simulink model "snap_sys_clk_feng"  (R2019a)
settings: Solver=VariableStepDiscrete  StartTime=0.0  StopTime=10.0  RelTol=1e-3
undefined symbols (not defined in the file): datetime, posixtime
libraries: xbsIndex_r4 x5252, casper_library_misc x69, xps_library x6, casper_library_delays x3
(part 12 of 45)

== system snap_sys_clk_feng/stats/calc_adc_sum_sq10 ==
  note: 127^2 == 16129
  in : Inport
  Accumulator : xbsIndex_r4/Accumulator  operation=Add  n_bits=32  overflow=Wrap  scale=1  rst=on  hasbypass=on  infoeditControl=reset for floating point data type must be asserted for a minimum of 2 cycles  en=off  latency=1  msb_inp=100  msb=100  lsb=-100  use_behavioral_HDL=on  implementation=Fabric  dbl_ovrd=off  block_type=accum
      settings: xl_area=[0, 0, 0, 0, 0, 0, 0]  block_version=10.1.3
  Accumulator1 : xbsIndex_r4/Accumulator  operation=Add  n_bits=32  overflow=Wrap  scale=1  rst=on  hasbypass=on  infoeditControl=reset for floating point data type must be asserted for a minimum of 2 cycles  en=off  latency=1  msb_inp=100  msb=100  lsb=-100  use_behavioral_HDL=on  implementation=Fabric  dbl_ovrd=off  block_type=accum
      settings: xl_area=[0, 0, 0, 0, 0, 0, 0]  block_version=10.1.3
  Accumulator2 : xbsIndex_r4/Accumulator  operation=Add  n_bits=32  overflow=Wrap  scale=1  rst=on  hasbypass=on  infoeditControl=reset for floating point data type must be asserted for a minimum of 2 cycles  en=off  latency=1  msb_inp=100  msb=100  lsb=-100  use_behavioral_HDL=on  implementation=Fabric  dbl_ovrd=off  block_type=accum
      settings: xl_area=[0, 0, 0, 0, 0, 0, 0]  block_version=10.1.3
  BitBasher : xbsIndex_r4/BitBasher  bitexpr=sss={clip, s, ss}  display_expr=off  sr_1=sss  arith_type1="Signed  (2's comp)"  bin_pt1=0  sr_2=2  arith_type2=Unsigned  bin_pt2=0  sr_3=3  arith_type3=Unsigned  bin_pt3=0  sr_4=4  arith_type4=Unsigned  bin_pt4=0  dbl_ovrd=off  block_type=bitbasher
      settings: block_version=10.1.3
  Constant : xbsIndex_r4/Constant  const=127^2  gui_display_data_type=Fixed-point  arith_type=Unsigned  n_bits=15  bin_pt=0  preci_type=Single  exp_width=8  frac_width=24  explicit_period=on  period=1  equ=P=C  opselect=C  inp2=PCIN>>17  opr=+  inp1=P  carry=CIN  dbl_ovrd=off  block_type=constant
  Delay : xbsIndex_r4/Delay  rst=off  infoeditControl=Selection of Reset will increase slice count due to use of real FFs and instead of SRLs  en=off  latency=2  reg_retiming=off  dbl_ovrd=off  block_type=delay
  Delay1 : xbsIndex_r4/Delay  rst=off  infoeditControl=Selection of Reset will increase slice count due to use of real FFs and instead of SRLs  en=off  latency=1  reg_retiming=off  dbl_ovrd=off  block_type=delay
  Delay2 : xbsIndex_r4/Delay  rst=off  infoeditControl=Selection of Reset will increase slice count due to use of real FFs and instead of SRLs  en=off  latency=1  reg_retiming=off  dbl_ovrd=off  block_type=delay
      settings: infoedit=Hardware notes: A delay line is a chain, each link of which is an SRL16 or SRL32 followed by a flip-flop.
  Mult : xbsIndex_r4/Mult  precision=User Defined  arith_type=Unsigned  n_bits=15  bin_pt=0  quantization=Truncate  overflow=Wrap  en=off  latency=2  use_behavioral_HDL=on  opt=Speed  use_embedded=on  optimum_pipeline=on  pipeline=on  dbl_ovrd=off  use_rpm=on  placement_style=Rectangular shape  block_type=mult
      settings: xl_area=[0, 0, 0, 0, 0, 0, 0]  block_version=10.1.3
  Register : xbsIndex_r4/Register  init=0  rst=off  en=on  dbl_ovrd=off  block_type=register
      settings: xl_area=[0, 0, 0, 0, 0, 0, 0]
  Register1 : xbsIndex_r4/Register  init=0  rst=off  en=on  dbl_ovrd=off  block_type=register
      settings: xl_area=[0, 0, 0, 0, 0, 0, 0]
  Register2 : xbsIndex_r4/Register  init=0  rst=off  en=on  dbl_ovrd=off  block_type=register
      settings: xl_area=[0, 0, 0, 0, 0, 0, 0]
  Reinterpret : xbsIndex_r4/Reinterpret  force_arith_type=off  arith_type=Unsigned  force_bin_pt=on  bin_pt=0  block_type=reinterpret
  Relational : xbsIndex_r4/Relational  mode=a>=b  op_type=Ufix  en=off  latency=0  dbl_ovrd=off  block_type=relational
  sum_sumsq : Outport
  wires:
  in/1 -> Reinterpret/1
  [adc_rms_rst] -> Delay2/1
  Accumulator/1 -> Register/1
  Mult/1 -> Accumulator/1, Relational/1
  Accumulator1/1 -> Register1/1
  Delay/1 -> Accumulator1/1
  BitBasher/1 -> sum_sumsq/1
  Delay1/1 -> Mult/2, Mult/1, Delay/1
  Reinterpret/1 -> Delay1/1
  Constant/1 -> Relational/2
  Relational/1 -> Accumulator2/1
  Delay2/1 -> Accumulator2/2, Accumulator1/2, Accumulator/2, Register2/2, Register1/2, Register/2
  Accumulator2/1 -> Register2/1
  Register1/1 -> BitBasher/2
  Register/1 -> BitBasher/3
  Register2/1 -> BitBasher/1

== system snap_sys_clk_feng/stats/calc_adc_sum_sq11 ==
  note: 127^2 == 16129
  in : Inport
  Accumulator : xbsIndex_r4/Accumulator  operation=Add  n_bits=32  overflow=Wrap  scale=1  rst=on  hasbypass=on  infoeditControl=reset for floating point data type must be asserted for a minimum of 2 cycles  en=off  latency=1  msb_inp=100  msb=100  lsb=-100  use_behavioral_HDL=on  implementation=Fabric  dbl_ovrd=off  block_type=accum
      settings: xl_area=[0, 0, 0, 0, 0, 0, 0]  block_version=10.1.3
  Accumulator1 : xbsIndex_r4/Accumulator  operation=Add  n_bits=32  overflow=Wrap  scale=1  rst=on  hasbypass=on  infoeditControl=reset for floating point data type must be asserted for a minimum of 2 cycles  en=off  latency=1  msb_inp=100  msb=100  lsb=-100  use_behavioral_HDL=on  implementation=Fabric  dbl_ovrd=off  block_type=accum
      settings: xl_area=[0, 0, 0, 0, 0, 0, 0]  block_version=10.1.3
  Accumulator2 : xbsIndex_r4/Accumulator  operation=Add  n_bits=32  overflow=Wrap  scale=1  rst=on  hasbypass=on  infoeditControl=reset for floating point data type must be asserted for a minimum of 2 cycles  en=off  latency=1  msb_inp=100  msb=100  lsb=-100  use_behavioral_HDL=on  implementation=Fabric  dbl_ovrd=off  block_type=accum
      settings: xl_area=[0, 0, 0, 0, 0, 0, 0]  block_version=10.1.3
  BitBasher : xbsIndex_r4/BitBasher  bitexpr=sss={clip, s, ss}  display_expr=off  sr_1=sss  arith_type1="Signed  (2's comp)"  bin_pt1=0  sr_2=2  arith_type2=Unsigned  bin_pt2=0  sr_3=3  arith_type3=Unsigned  bin_pt3=0  sr_4=4  arith_type4=Unsigned  bin_pt4=0  dbl_ovrd=off  block_type=bitbasher
      settings: block_version=10.1.3
  Constant : xbsIndex_r4/Constant  const=127^2  gui_display_data_type=Fixed-point  arith_type=Unsigned  n_bits=15  bin_pt=0  preci_type=Single  exp_width=8  frac_width=24  explicit_period=on  period=1  equ=P=C  opselect=C  inp2=PCIN>>17  opr=+  inp1=P  carry=CIN  dbl_ovrd=off  block_type=constant
  Delay : xbsIndex_r4/Delay  rst=off  infoeditControl=Selection of Reset will increase slice count due to use of real FFs and instead of SRLs  en=off  latency=2  reg_retiming=off  dbl_ovrd=off  block_type=delay
  Delay1 : xbsIndex_r4/Delay  rst=off  infoeditControl=Selection of Reset will increase slice count due to use of real FFs and instead of SRLs  en=off  latency=1  reg_retiming=off  dbl_ovrd=off  block_type=delay
  Delay2 : xbsIndex_r4/Delay  rst=off  infoeditControl=Selection of Reset will increase slice count due to use of real FFs and instead of SRLs  en=off  latency=1  reg_retiming=off  dbl_ovrd=off  block_type=delay
      settings: infoedit=Hardware notes: A delay line is a chain, each link of which is an SRL16 or SRL32 followed by a flip-flop.
  Mult : xbsIndex_r4/Mult  precision=User Defined  arith_type=Unsigned  n_bits=15  bin_pt=0  quantization=Truncate  overflow=Wrap  en=off  latency=2  use_behavioral_HDL=on  opt=Speed  use_embedded=on  optimum_pipeline=on  pipeline=on  dbl_ovrd=off  use_rpm=on  placement_style=Rectangular shape  block_type=mult
      settings: xl_area=[0, 0, 0, 0, 0, 0, 0]  block_version=10.1.3
  Register : xbsIndex_r4/Register  init=0  rst=off  en=on  dbl_ovrd=off  block_type=register
      settings: xl_area=[0, 0, 0, 0, 0, 0, 0]
  Register1 : xbsIndex_r4/Register  init=0  rst=off  en=on  dbl_ovrd=off  block_type=register
      settings: xl_area=[0, 0, 0, 0, 0, 0, 0]
  Register2 : xbsIndex_r4/Register  init=0  rst=off  en=on  dbl_ovrd=off  block_type=register
      settings: xl_area=[0, 0, 0, 0, 0, 0, 0]
  Reinterpret : xbsIndex_r4/Reinterpret  force_arith_type=off  arith_type=Unsigned  force_bin_pt=on  bin_pt=0  block_type=reinterpret
  Relational : xbsIndex_r4/Relational  mode=a>=b  op_type=Ufix  en=off  latency=0  dbl_ovrd=off  block_type=relational
  sum_sumsq : Outport
  wires:
  Register2/1 -> BitBasher/1
  Register/1 -> BitBasher/3
  Register1/1 -> BitBasher/2
  Accumulator2/1 -> Register2/1
  Delay2/1 -> Register/2, Register1/2, Register2/2, Accumulator/2, Accumulator1/2, Accumulator2/2
  Relational/1 -> Accumulator2/1
  Constant/1 -> Relational/2
  Reinterpret/1 -> Delay1/1
  Delay1/1 -> Delay/1, Mult/1, Mult/2
  BitBasher/1 -> sum_sumsq/1
  Delay/1 -> Accumulator1/1
  Accumulator1/1 -> Register1/1
  Mult/1 -> Relational/1, Accumulator/1
  Accumulator/1 -> Register/1
  [adc_rms_rst] -> Delay2/1
  in/1 -> Reinterpret/1

== system snap_sys_clk_feng/stats/calc_adc_sum_sq12 ==
  note: 127^2 == 16129
  in : Inport
  Accumulator : xbsIndex_r4/Accumulator  operation=Add  n_bits=32  overflow=Wrap  scale=1  rst=on  hasbypass=on  infoeditControl=reset for floating point data type must be asserted for a minimum of 2 cycles  en=off  latency=1  msb_inp=100  msb=100  lsb=-100  use_behavioral_HDL=on  implementation=Fabric  dbl_ovrd=off  block_type=accum
      settings: xl_area=[0, 0, 0, 0, 0, 0, 0]  block_version=10.1.3
  Accumulator1 : xbsIndex_r4/Accumulator  operation=Add  n_bits=32  overflow=Wrap  scale=1  rst=on  hasbypass=on  infoeditControl=reset for floating point data type must be asserted for a minimum of 2 cycles  en=off  latency=1  msb_inp=100  msb=100  lsb=-100  use_behavioral_HDL=on  implementation=Fabric  dbl_ovrd=off  block_type=accum
      settings: xl_area=[0, 0, 0, 0, 0, 0, 0]  block_version=10.1.3
  Accumulator2 : xbsIndex_r4/Accumulator  operation=Add  n_bits=32  overflow=Wrap  scale=1  rst=on  hasbypass=on  infoeditControl=reset for floating point data type must be asserted for a minimum of 2 cycles  en=off  latency=1  msb_inp=100  msb=100  lsb=-100  use_behavioral_HDL=on  implementation=Fabric  dbl_ovrd=off  block_type=accum
      settings: xl_area=[0, 0, 0, 0, 0, 0, 0]  block_version=10.1.3
  BitBasher : xbsIndex_r4/BitBasher  bitexpr=sss={clip, s, ss}  display_expr=off  sr_1=sss  arith_type1="Signed  (2's comp)"  bin_pt1=0  sr_2=2  arith_type2=Unsigned  bin_pt2=0  sr_3=3  arith_type3=Unsigned  bin_pt3=0  sr_4=4  arith_type4=Unsigned  bin_pt4=0  dbl_ovrd=off  block_type=bitbasher
      settings: block_version=10.1.3
  Constant : xbsIndex_r4/Constant  const=127^2  gui_display_data_type=Fixed-point  arith_type=Unsigned  n_bits=15  bin_pt=0  preci_type=Single  exp_width=8  frac_width=24  explicit_period=on  period=1  equ=P=C  opselect=C  inp2=PCIN>>17  opr=+  inp1=P  carry=CIN  dbl_ovrd=off  block_type=constant
  Delay : xbsIndex_r4/Delay  rst=off  infoeditControl=Selection of Reset will increase slice count due to use of real FFs and instead of SRLs  en=off  latency=2  reg_retiming=off  dbl_ovrd=off  block_type=delay
  Delay1 : xbsIndex_r4/Delay  rst=off  infoeditControl=Selection of Reset will increase slice count due to use of real FFs and instead of SRLs  en=off  latency=1  reg_retiming=off  dbl_ovrd=off  block_type=delay
  Delay2 : xbsIndex_r4/Delay  rst=off  infoeditControl=Selection of Reset will increase slice count due to use of real FFs and instead of SRLs  en=off  latency=1  reg_retiming=off  dbl_ovrd=off  block_type=delay
      settings: infoedit=Hardware notes: A delay line is a chain, each link of which is an SRL16 or SRL32 followed by a flip-flop.
  Mult : xbsIndex_r4/Mult  precision=User Defined  arith_type=Unsigned  n_bits=15  bin_pt=0  quantization=Truncate  overflow=Wrap  en=off  latency=2  use_behavioral_HDL=on  opt=Speed  use_embedded=on  optimum_pipeline=on  pipeline=on  dbl_ovrd=off  use_rpm=on  placement_style=Rectangular shape  block_type=mult
      settings: xl_area=[0, 0, 0, 0, 0, 0, 0]  block_version=10.1.3
  Register : xbsIndex_r4/Register  init=0  rst=off  en=on  dbl_ovrd=off  block_type=register
      settings: xl_area=[0, 0, 0, 0, 0, 0, 0]
  Register1 : xbsIndex_r4/Register  init=0  rst=off  en=on  dbl_ovrd=off  block_type=register
      settings: xl_area=[0, 0, 0, 0, 0, 0, 0]
  Register2 : xbsIndex_r4/Register  init=0  rst=off  en=on  dbl_ovrd=off  block_type=register
      settings: xl_area=[0, 0, 0, 0, 0, 0, 0]
  Reinterpret : xbsIndex_r4/Reinterpret  force_arith_type=off  arith_type=Unsigned  force_bin_pt=on  bin_pt=0  block_type=reinterpret
  Relational : xbsIndex_r4/Relational  mode=a>=b  op_type=Ufix  en=off  latency=0  dbl_ovrd=off  block_type=relational
  sum_sumsq : Outport
  wires:
  in/1 -> Reinterpret/1
  [adc_rms_rst] -> Delay2/1
  Accumulator/1 -> Register/1
  Mult/1 -> Accumulator/1, Relational/1
  Accumulator1/1 -> Register1/1
  Delay/1 -> Accumulator1/1
  BitBasher/1 -> sum_sumsq/1
  Delay1/1 -> Mult/2, Mult/1, Delay/1
  Reinterpret/1 -> Delay1/1
  Constant/1 -> Relational/2
  Relational/1 -> Accumulator2/1
  Delay2/1 -> Accumulator2/2, Accumulator1/2, Accumulator/2, Register2/2, Register1/2, Register/2
  Accumulator2/1 -> Register2/1
  Register1/1 -> BitBasher/2
  Register/1 -> BitBasher/3
  Register2/1 -> BitBasher/1

== system snap_sys_clk_feng/stats/calc_adc_sum_sq13 ==
  note: 127^2 == 16129
  in : Inport
  Accumulator : xbsIndex_r4/Accumulator  operation=Add  n_bits=32  overflow=Wrap  scale=1  rst=on  hasbypass=on  infoeditControl=reset for floating point data type must be asserted for a minimum of 2 cycles  en=off  latency=1  msb_inp=100  msb=100  lsb=-100  use_behavioral_HDL=on  implementation=Fabric  dbl_ovrd=off  block_type=accum
      settings: xl_area=[0, 0, 0, 0, 0, 0, 0]  block_version=10.1.3
  Accumulator1 : xbsIndex_r4/Accumulator  operation=Add  n_bits=32  overflow=Wrap  scale=1  rst=on  hasbypass=on  infoeditControl=reset for floating point data type must be asserted for a minimum of 2 cycles  en=off  latency=1  msb_inp=100  msb=100  lsb=-100  use_behavioral_HDL=on  implementation=Fabric  dbl_ovrd=off  block_type=accum
      settings: xl_area=[0, 0, 0, 0, 0, 0, 0]  block_version=10.1.3
  Accumulator2 : xbsIndex_r4/Accumulator  operation=Add  n_bits=32  overflow=Wrap  scale=1  rst=on  hasbypass=on  infoeditControl=reset for floating point data type must be asserted for a minimum of 2 cycles  en=off  latency=1  msb_inp=100  msb=100  lsb=-100  use_behavioral_HDL=on  implementation=Fabric  dbl_ovrd=off  block_type=accum
      settings: xl_area=[0, 0, 0, 0, 0, 0, 0]  block_version=10.1.3
  BitBasher : xbsIndex_r4/BitBasher  bitexpr=sss={clip, s, ss}  display_expr=off  sr_1=sss  arith_type1="Signed  (2's comp)"  bin_pt1=0  sr_2=2  arith_type2=Unsigned  bin_pt2=0  sr_3=3  arith_type3=Unsigned  bin_pt3=0  sr_4=4  arith_type4=Unsigned  bin_pt4=0  dbl_ovrd=off  block_type=bitbasher
      settings: block_version=10.1.3
  Constant : xbsIndex_r4/Constant  const=127^2  gui_display_data_type=Fixed-point  arith_type=Unsigned  n_bits=15  bin_pt=0  preci_type=Single  exp_width=8  frac_width=24  explicit_period=on  period=1  equ=P=C  opselect=C  inp2=PCIN>>17  opr=+  inp1=P  carry=CIN  dbl_ovrd=off  block_type=constant
  Delay : xbsIndex_r4/Delay  rst=off  infoeditControl=Selection of Reset will increase slice count due to use of real FFs and instead of SRLs  en=off  latency=2  reg_retiming=off  dbl_ovrd=off  block_type=delay
  Delay1 : xbsIndex_r4/Delay  rst=off  infoeditControl=Selection of Reset will increase slice count due to use of real FFs and instead of SRLs  en=off  latency=1  reg_retiming=off  dbl_ovrd=off  block_type=delay
  Delay2 : xbsIndex_r4/Delay  rst=off  infoeditControl=Selection of Reset will increase slice count due to use of real FFs and instead of SRLs  en=off  latency=1  reg_retiming=off  dbl_ovrd=off  block_type=delay
      settings: infoedit=Hardware notes: A delay line is a chain, each link of which is an SRL16 or SRL32 followed by a flip-flop.
  Mult : xbsIndex_r4/Mult  precision=User Defined  arith_type=Unsigned  n_bits=15  bin_pt=0  quantization=Truncate  overflow=Wrap  en=off  latency=2  use_behavioral_HDL=on  opt=Speed  use_embedded=on  optimum_pipeline=on  pipeline=on  dbl_ovrd=off  use_rpm=on  placement_style=Rectangular shape  block_type=mult
      settings: xl_area=[0, 0, 0, 0, 0, 0, 0]  block_version=10.1.3
  Register : xbsIndex_r4/Register  init=0  rst=off  en=on  dbl_ovrd=off  block_type=register
      settings: xl_area=[0, 0, 0, 0, 0, 0, 0]
  Register1 : xbsIndex_r4/Register  init=0  rst=off  en=on  dbl_ovrd=off  block_type=register
      settings: xl_area=[0, 0, 0, 0, 0, 0, 0]
  Register2 : xbsIndex_r4/Register  init=0  rst=off  en=on  dbl_ovrd=off  block_type=register
      settings: xl_area=[0, 0, 0, 0, 0, 0, 0]
  Reinterpret : xbsIndex_r4/Reinterpret  force_arith_type=off  arith_type=Unsigned  force_bin_pt=on  bin_pt=0  block_type=reinterpret
  Relational : xbsIndex_r4/Relational  mode=a>=b  op_type=Ufix  en=off  latency=0  dbl_ovrd=off  block_type=relational
  sum_sumsq : Outport
  wires:
  Register2/1 -> BitBasher/1
  Register/1 -> BitBasher/3
  Register1/1 -> BitBasher/2
  Accumulator2/1 -> Register2/1
  Delay2/1 -> Register/2, Register1/2, Register2/2, Accumulator/2, Accumulator1/2, Accumulator2/2
  Relational/1 -> Accumulator2/1
  Constant/1 -> Relational/2
  Reinterpret/1 -> Delay1/1
  Delay1/1 -> Delay/1, Mult/1, Mult/2
  BitBasher/1 -> sum_sumsq/1
  Delay/1 -> Accumulator1/1
  Accumulator1/1 -> Register1/1
  Mult/1 -> Relational/1, Accumulator/1
  Accumulator/1 -> Register/1
  [adc_rms_rst] -> Delay2/1
  in/1 -> Reinterpret/1

== system snap_sys_clk_feng/stats/calc_adc_sum_sq14 ==
  note: 127^2 == 16129
  in : Inport
  Accumulator : xbsIndex_r4/Accumulator  operation=Add  n_bits=32  overflow=Wrap  scale=1  rst=on  hasbypass=on  infoeditControl=reset for floating point data type must be asserted for a minimum of 2 cycles  en=off  latency=1  msb_inp=100  msb=100  lsb=-100  use_behavioral_HDL=on  implementation=Fabric  dbl_ovrd=off  block_type=accum
      settings: xl_area=[0, 0, 0, 0, 0, 0, 0]  block_version=10.1.3
  Accumulator1 : xbsIndex_r4/Accumulator  operation=Add  n_bits=32  overflow=Wrap  scale=1  rst=on  hasbypass=on  infoeditControl=reset for floating point data type must be asserted for a minimum of 2 cycles  en=off  latency=1  msb_inp=100  msb=100  lsb=-100  use_behavioral_HDL=on  implementation=Fabric  dbl_ovrd=off  block_type=accum
      settings: xl_area=[0, 0, 0, 0, 0, 0, 0]  block_version=10.1.3
  Accumulator2 : xbsIndex_r4/Accumulator  operation=Add  n_bits=32  overflow=Wrap  scale=1  rst=on  hasbypass=on  infoeditControl=reset for floating point data type must be asserted for a minimum of 2 cycles  en=off  latency=1  msb_inp=100  msb=100  lsb=-100  use_behavioral_HDL=on  implementation=Fabric  dbl_ovrd=off  block_type=accum
      settings: xl_area=[0, 0, 0, 0, 0, 0, 0]  block_version=10.1.3
  BitBasher : xbsIndex_r4/BitBasher  bitexpr=sss={clip, s, ss}  display_expr=off  sr_1=sss  arith_type1="Signed  (2's comp)"  bin_pt1=0  sr_2=2  arith_type2=Unsigned  bin_pt2=0  sr_3=3  arith_type3=Unsigned  bin_pt3=0  sr_4=4  arith_type4=Unsigned  bin_pt4=0  dbl_ovrd=off  block_type=bitbasher
      settings: block_version=10.1.3
  Constant : xbsIndex_r4/Constant  const=127^2  gui_display_data_type=Fixed-point  arith_type=Unsigned  n_bits=15  bin_pt=0  preci_type=Single  exp_width=8  frac_width=24  explicit_period=on  period=1  equ=P=C  opselect=C  inp2=PCIN>>17  opr=+  inp1=P  carry=CIN  dbl_ovrd=off  block_type=constant
  Delay : xbsIndex_r4/Delay  rst=off  infoeditControl=Selection of Reset will increase slice count due to use of real FFs and instead of SRLs  en=off  latency=2  reg_retiming=off  dbl_ovrd=off  block_type=delay
  Delay1 : xbsIndex_r4/Delay  rst=off  infoeditControl=Selection of Reset will increase slice count due to use of real FFs and instead of SRLs  en=off  latency=1  reg_retiming=off  dbl_ovrd=off  block_type=delay
  Delay2 : xbsIndex_r4/Delay  rst=off  infoeditControl=Selection of Reset will increase slice count due to use of real FFs and instead of SRLs  en=off  latency=1  reg_retiming=off  dbl_ovrd=off  block_type=delay
      settings: infoedit=Hardware notes: A delay line is a chain, each link of which is an SRL16 or SRL32 followed by a flip-flop.
  Mult : xbsIndex_r4/Mult  precision=User Defined  arith_type=Unsigned  n_bits=15  bin_pt=0  quantization=Truncate  overflow=Wrap  en=off  latency=2  use_behavioral_HDL=on  opt=Speed  use_embedded=on  optimum_pipeline=on  pipeline=on  dbl_ovrd=off  use_rpm=on  placement_style=Rectangular shape  block_type=mult
      settings: xl_area=[0, 0, 0, 0, 0, 0, 0]  block_version=10.1.3
  Register : xbsIndex_r4/Register  init=0  rst=off  en=on  dbl_ovrd=off  block_type=register
      settings: xl_area=[0, 0, 0, 0, 0, 0, 0]
  Register1 : xbsIndex_r4/Register  init=0  rst=off  en=on  dbl_ovrd=off  block_type=register
      settings: xl_area=[0, 0, 0, 0, 0, 0, 0]
  Register2 : xbsIndex_r4/Register  init=0  rst=off  en=on  dbl_ovrd=off  block_type=register
      settings: xl_area=[0, 0, 0, 0, 0, 0, 0]
  Reinterpret : xbsIndex_r4/Reinterpret  force_arith_type=off  arith_type=Unsigned  force_bin_pt=on  bin_pt=0  block_type=reinterpret
  Relational : xbsIndex_r4/Relational  mode=a>=b  op_type=Ufix  en=off  latency=0  dbl_ovrd=off  block_type=relational
  sum_sumsq : Outport
  wires:
  Register2/1 -> BitBasher/1
  Register/1 -> BitBasher/3
  Register1/1 -> BitBasher/2
  Accumulator2/1 -> Register2/1
  Delay2/1 -> Register/2, Register1/2, Register2/2, Accumulator/2, Accumulator1/2, Accumulator2/2
  Relational/1 -> Accumulator2/1
  Constant/1 -> Relational/2
  Reinterpret/1 -> Delay1/1
  Delay1/1 -> Delay/1, Mult/1, Mult/2
  BitBasher/1 -> sum_sumsq/1
  Delay/1 -> Accumulator1/1
  Accumulator1/1 -> Register1/1
  Mult/1 -> Relational/1, Accumulator/1
  Accumulator/1 -> Register/1
  [adc_rms_rst] -> Delay2/1
  in/1 -> Reinterpret/1

== system snap_sys_clk_feng/stats/calc_adc_sum_sq15 ==
  note: 127^2 == 16129
  in : Inport
  Accumulator : xbsIndex_r4/Accumulator  operation=Add  n_bits=32  overflow=Wrap  scale=1  rst=on  hasbypass=on  infoeditControl=reset for floating point data type must be asserted for a minimum of 2 cycles  en=off  latency=1  msb_inp=100  msb=100  lsb=-100  use_behavioral_HDL=on  implementation=Fabric  dbl_ovrd=off  block_type=accum
      settings: xl_area=[0, 0, 0, 0, 0, 0, 0]  block_version=10.1.3
  Accumulator1 : xbsIndex_r4/Accumulator  operation=Add  n_bits=32  overflow=Wrap  scale=1  rst=on  hasbypass=on  infoeditControl=reset for floating point data type must be asserted for a minimum of 2 cycles  en=off  latency=1  msb_inp=100  msb=100  lsb=-100  use_behavioral_HDL=on  implementation=Fabric  dbl_ovrd=off  block_type=accum
      settings: xl_area=[0, 0, 0, 0, 0, 0, 0]  block_version=10.1.3
  Accumulator2 : xbsIndex_r4/Accumulator  operation=Add  n_bits=32  overflow=Wrap  scale=1  rst=on  hasbypass=on  infoeditControl=reset for floating point data type must be asserted for a minimum of 2 cycles  en=off  latency=1  msb_inp=100  msb=100  lsb=-100  use_behavioral_HDL=on  implementation=Fabric  dbl_ovrd=off  block_type=accum
      settings: xl_area=[0, 0, 0, 0, 0, 0, 0]  block_version=10.1.3
  BitBasher : xbsIndex_r4/BitBasher  bitexpr=sss={clip, s, ss}  display_expr=off  sr_1=sss  arith_type1="Signed  (2's comp)"  bin_pt1=0  sr_2=2  arith_type2=Unsigned  bin_pt2=0  sr_3=3  arith_type3=Unsigned  bin_pt3=0  sr_4=4  arith_type4=Unsigned  bin_pt4=0  dbl_ovrd=off  block_type=bitbasher
      settings: block_version=10.1.3
  Constant : xbsIndex_r4/Constant  const=127^2  gui_display_data_type=Fixed-point  arith_type=Unsigned  n_bits=15  bin_pt=0  preci_type=Single  exp_width=8  frac_width=24  explicit_period=on  period=1  equ=P=C  opselect=C  inp2=PCIN>>17  opr=+  inp1=P  carry=CIN  dbl_ovrd=off  block_type=constant
  Delay : xbsIndex_r4/Delay  rst=off  infoeditControl=Selection of Reset will increase slice count due to use of real FFs and instead of SRLs  en=off  latency=2  reg_retiming=off  dbl_ovrd=off  block_type=delay
  Delay1 : xbsIndex_r4/Delay  rst=off  infoeditControl=Selection of Reset will increase slice count due to use of real FFs and instead of SRLs  en=off  latency=1  reg_retiming=off  dbl_ovrd=off  block_type=delay
  Delay2 : xbsIndex_r4/Delay  rst=off  infoeditControl=Selection of Reset will increase slice count due to use of real FFs and instead of SRLs  en=off  latency=1  reg_retiming=off  dbl_ovrd=off  block_type=delay
      settings: infoedit=Hardware notes: A delay line is a chain, each link of which is an SRL16 or SRL32 followed by a flip-flop.
  Mult : xbsIndex_r4/Mult  precision=User Defined  arith_type=Unsigned  n_bits=15  bin_pt=0  quantization=Truncate  overflow=Wrap  en=off  latency=2  use_behavioral_HDL=on  opt=Speed  use_embedded=on  optimum_pipeline=on  pipeline=on  dbl_ovrd=off  use_rpm=on  placement_style=Rectangular shape  block_type=mult
      settings: xl_area=[0, 0, 0, 0, 0, 0, 0]  block_version=10.1.3
  Register : xbsIndex_r4/Register  init=0  rst=off  en=on  dbl_ovrd=off  block_type=register
      settings: xl_area=[0, 0, 0, 0, 0, 0, 0]
  Register1 : xbsIndex_r4/Register  init=0  rst=off  en=on  dbl_ovrd=off  block_type=register
      settings: xl_area=[0, 0, 0, 0, 0, 0, 0]
  Register2 : xbsIndex_r4/Register  init=0  rst=off  en=on  dbl_ovrd=off  block_type=register
      settings: xl_area=[0, 0, 0, 0, 0, 0, 0]
  Reinterpret : xbsIndex_r4/Reinterpret  force_arith_type=off  arith_type=Unsigned  force_bin_pt=on  bin_pt=0  block_type=reinterpret
  Relational : xbsIndex_r4/Relational  mode=a>=b  op_type=Ufix  en=off  latency=0  dbl_ovrd=off  block_type=relational
  sum_sumsq : Outport
  wires:
  in/1 -> Reinterpret/1
  [adc_rms_rst] -> Delay2/1
  Accumulator/1 -> Register/1
  Mult/1 -> Accumulator/1, Relational/1
  Accumulator1/1 -> Register1/1
  Delay/1 -> Accumulator1/1
  BitBasher/1 -> sum_sumsq/1
  Delay1/1 -> Mult/2, Mult/1, Delay/1
  Reinterpret/1 -> Delay1/1
  Constant/1 -> Relational/2
  Relational/1 -> Accumulator2/1
  Delay2/1 -> Accumulator2/2, Accumulator1/2, Accumulator/2, Register2/2, Register1/2, Register/2
  Accumulator2/1 -> Register2/1
  Register1/1 -> BitBasher/2
  Register/1 -> BitBasher/3
  Register2/1 -> BitBasher/1

== system snap_sys_clk_feng/stats/calc_adc_sum_sq2 ==
  note: 127^2 == 16129
  in : Inport
  Accumulator : xbsIndex_r4/Accumulator  operation=Add  n_bits=32  overflow=Wrap  scale=1  rst=on  hasbypass=on  infoeditControl=reset for floating point data type must be asserted for a minimum of 2 cycles  en=off  latency=1  msb_inp=100  msb=100  lsb=-100  use_behavioral_HDL=on  implementation=Fabric  dbl_ovrd=off  block_type=accum
      settings: xl_area=[0, 0, 0, 0, 0, 0, 0]  block_version=10.1.3
  Accumulator1 : xbsIndex_r4/Accumulator  operation=Add  n_bits=32  overflow=Wrap  scale=1  rst=on  hasbypass=on  infoeditControl=reset for floating point data type must be asserted for a minimum of 2 cycles  en=off  latency=1  msb_inp=100  msb=100  lsb=-100  use_behavioral_HDL=on  implementation=Fabric  dbl_ovrd=off  block_type=accum
      settings: xl_area=[0, 0, 0, 0, 0, 0, 0]  block_version=10.1.3
  Accumulator2 : xbsIndex_r4/Accumulator  operation=Add  n_bits=32  overflow=Wrap  scale=1  rst=on  hasbypass=on  infoeditControl=reset for floating point data type must be asserted for a minimum of 2 cycles  en=off  latency=1  msb_inp=100  msb=100  lsb=-100  use_behavioral_HDL=on  implementation=Fabric  dbl_ovrd=off  block_type=accum
      settings: xl_area=[0, 0, 0, 0, 0, 0, 0]  block_version=10.1.3
  BitBasher : xbsIndex_r4/BitBasher  bitexpr=sss={clip, s, ss}  display_expr=off  sr_1=sss  arith_type1="Signed  (2's comp)"  bin_pt1=0  sr_2=2  arith_type2=Unsigned  bin_pt2=0  sr_3=3  arith_type3=Unsigned  bin_pt3=0  sr_4=4  arith_type4=Unsigned  bin_pt4=0  dbl_ovrd=off  block_type=bitbasher
      settings: block_version=10.1.3
  Constant : xbsIndex_r4/Constant  const=127^2  gui_display_data_type=Fixed-point  arith_type=Unsigned  n_bits=15  bin_pt=0  preci_type=Single  exp_width=8  frac_width=24  explicit_period=on  period=1  equ=P=C  opselect=C  inp2=PCIN>>17  opr=+  inp1=P  carry=CIN  dbl_ovrd=off  block_type=constant
  Delay : xbsIndex_r4/Delay  rst=off  infoeditControl=Selection of Reset will increase slice count due to use of real FFs and instead of SRLs  en=off  latency=2  reg_retiming=off  dbl_ovrd=off  block_type=delay
  Delay1 : xbsIndex_r4/Delay  rst=off  infoeditControl=Selection of Reset will increase slice count due to use of real FFs and instead of SRLs  en=off  latency=1  reg_retiming=off  dbl_ovrd=off  block_type=delay
  Delay2 : xbsIndex_r4/Delay  rst=off  infoeditControl=Selection of Reset will increase slice count due to use of real FFs and instead of SRLs  en=off  latency=1  reg_retiming=off  dbl_ovrd=off  block_type=delay
      settings: infoedit=Hardware notes: A delay line is a chain, each link of which is an SRL16 or SRL32 followed by a flip-flop.
  Mult : xbsIndex_r4/Mult  precision=User Defined  arith_type=Unsigned  n_bits=15  bin_pt=0  quantization=Truncate  overflow=Wrap  en=off  latency=2  use_behavioral_HDL=on  opt=Speed  use_embedded=on  optimum_pipeline=on  pipeline=on  dbl_ovrd=off  use_rpm=on  placement_style=Rectangular shape  block_type=mult
      settings: xl_area=[0, 0, 0, 0, 0, 0, 0]  block_version=10.1.3
  Register : xbsIndex_r4/Register  init=0  rst=off  en=on  dbl_ovrd=off  block_type=register
      settings: xl_area=[0, 0, 0, 0, 0, 0, 0]
  Register1 : xbsIndex_r4/Register  init=0  rst=off  en=on  dbl_ovrd=off  block_type=register
      settings: xl_area=[0, 0, 0, 0, 0, 0, 0]
  Register2 : xbsIndex_r4/Register  init=0  rst=off  en=on  dbl_ovrd=off  block_type=register
      settings: xl_area=[0, 0, 0, 0, 0, 0, 0]
  Reinterpret : xbsIndex_r4/Reinterpret  force_arith_type=off  arith_type=Unsigned  force_bin_pt=on  bin_pt=0  block_type=reinterpret
  Relational : xbsIndex_r4/Relational  mode=a>=b  op_type=Ufix  en=off  latency=0  dbl_ovrd=off  block_type=relational
  sum_sumsq : Outport
  wires:
  Register2/1 -> BitBasher/1
  Register/1 -> BitBasher/3
  Register1/1 -> BitBasher/2
  Accumulator2/1 -> Register2/1
  Delay2/1 -> Register/2, Register1/2, Register2/2, Accumulator/2, Accumulator1/2, Accumulator2/2
  Relational/1 -> Accumulator2/1
  Constant/1 -> Relational/2
  Reinterpret/1 -> Delay1/1
  Delay1/1 -> Delay/1, Mult/1, Mult/2
  BitBasher/1 -> sum_sumsq/1
  Delay/1 -> Accumulator1/1
  Accumulator1/1 -> Register1/1
  Mult/1 -> Relational/1, Accumulator/1
  Accumulator/1 -> Register/1
  [adc_rms_rst] -> Delay2/1
  in/1 -> Reinterpret/1

== system snap_sys_clk_feng/stats/calc_adc_sum_sq3 ==
  note: 127^2 == 16129
  in : Inport
  Accumulator : xbsIndex_r4/Accumulator  operation=Add  n_bits=32  overflow=Wrap  scale=1  rst=on  hasbypass=on  infoeditControl=reset for floating point data type must be asserted for a minimum of 2 cycles  en=off  latency=1  msb_inp=100  msb=100  lsb=-100  use_behavioral_HDL=on  implementation=Fabric  dbl_ovrd=off  block_type=accum
      settings: xl_area=[0, 0, 0, 0, 0, 0, 0]  block_version=10.1.3
  Accumulator1 : xbsIndex_r4/Accumulator  operation=Add  n_bits=32  overflow=Wrap  scale=1  rst=on  hasbypass=on  infoeditControl=reset for floating point data type must be asserted for a minimum of 2 cycles  en=off  latency=1  msb_inp=100  msb=100  lsb=-100  use_behavioral_HDL=on  implementation=Fabric  dbl_ovrd=off  block_type=accum
      settings: xl_area=[0, 0, 0, 0, 0, 0, 0]  block_version=10.1.3
  Accumulator2 : xbsIndex_r4/Accumulator  operation=Add  n_bits=32  overflow=Wrap  scale=1  rst=on  hasbypass=on  infoeditControl=reset for floating point data type must be asserted for a minimum of 2 cycles  en=off  latency=1  msb_inp=100  msb=100  lsb=-100  use_behavioral_HDL=on  implementation=Fabric  dbl_ovrd=off  block_type=accum
      settings: xl_area=[0, 0, 0, 0, 0, 0, 0]  block_version=10.1.3
  BitBasher : xbsIndex_r4/BitBasher  bitexpr=sss={clip, s, ss}  display_expr=off  sr_1=sss  arith_type1="Signed  (2's comp)"  bin_pt1=0  sr_2=2  arith_type2=Unsigned  bin_pt2=0  sr_3=3  arith_type3=Unsigned  bin_pt3=0  sr_4=4  arith_type4=Unsigned  bin_pt4=0  dbl_ovrd=off  block_type=bitbasher
      settings: block_version=10.1.3
  Constant : xbsIndex_r4/Constant  const=127^2  gui_display_data_type=Fixed-point  arith_type=Unsigned  n_bits=15  bin_pt=0  preci_type=Single  exp_width=8  frac_width=24  explicit_period=on  period=1  equ=P=C  opselect=C  inp2=PCIN>>17  opr=+  inp1=P  carry=CIN  dbl_ovrd=off  block_type=constant
  Delay : xbsIndex_r4/Delay  rst=off  infoeditControl=Selection of Reset will increase slice count due to use of real FFs and instead of SRLs  en=off  latency=2  reg_retiming=off  dbl_ovrd=off  block_type=delay
  Delay1 : xbsIndex_r4/Delay  rst=off  infoeditControl=Selection of Reset will increase slice count due to use of real FFs and instead of SRLs  en=off  latency=1  reg_retiming=off  dbl_ovrd=off  block_type=delay
  Delay2 : xbsIndex_r4/Delay  rst=off  infoeditControl=Selection of Reset will increase slice count due to use of real FFs and instead of SRLs  en=off  latency=1  reg_retiming=off  dbl_ovrd=off  block_type=delay
      settings: infoedit=Hardware notes: A delay line is a chain, each link of which is an SRL16 or SRL32 followed by a flip-flop.
  Mult : xbsIndex_r4/Mult  precision=User Defined  arith_type=Unsigned  n_bits=15  bin_pt=0  quantization=Truncate  overflow=Wrap  en=off  latency=2  use_behavioral_HDL=on  opt=Speed  use_embedded=on  optimum_pipeline=on  pipeline=on  dbl_ovrd=off  use_rpm=on  placement_style=Rectangular shape  block_type=mult
      settings: xl_area=[0, 0, 0, 0, 0, 0, 0]  block_version=10.1.3
  Register : xbsIndex_r4/Register  init=0  rst=off  en=on  dbl_ovrd=off  block_type=register
      settings: xl_area=[0, 0, 0, 0, 0, 0, 0]
  Register1 : xbsIndex_r4/Register  init=0  rst=off  en=on  dbl_ovrd=off  block_type=register
      settings: xl_area=[0, 0, 0, 0, 0, 0, 0]
  Register2 : xbsIndex_r4/Register  init=0  rst=off  en=on  dbl_ovrd=off  block_type=register
      settings: xl_area=[0, 0, 0, 0, 0, 0, 0]
  Reinterpret : xbsIndex_r4/Reinterpret  force_arith_type=off  arith_type=Unsigned  force_bin_pt=on  bin_pt=0  block_type=reinterpret
  Relational : xbsIndex_r4/Relational  mode=a>=b  op_type=Ufix  en=off  latency=0  dbl_ovrd=off  block_type=relational
  sum_sumsq : Outport
  wires:
  in/1 -> Reinterpret/1
  [adc_rms_rst] -> Delay2/1
  Accumulator/1 -> Register/1
  Mult/1 -> Accumulator/1, Relational/1
  Accumulator1/1 -> Register1/1
  Delay/1 -> Accumulator1/1
  BitBasher/1 -> sum_sumsq/1
  Delay1/1 -> Mult/2, Mult/1, Delay/1
  Reinterpret/1 -> Delay1/1
  Constant/1 -> Relational/2
  Relational/1 -> Accumulator2/1
  Delay2/1 -> Accumulator2/2, Accumulator1/2, Accumulator/2, Register2/2, Register1/2, Register/2
  Accumulator2/1 -> Register2/1
  Register1/1 -> BitBasher/2
  Register/1 -> BitBasher/3
  Register2/1 -> BitBasher/1

== system snap_sys_clk_feng/stats/calc_adc_sum_sq4 ==
  note: 127^2 == 16129
  in : Inport
  Accumulator : xbsIndex_r4/Accumulator  operation=Add  n_bits=32  overflow=Wrap  scale=1  rst=on  hasbypass=on  infoeditControl=reset for floating point data type must be asserted for a minimum of 2 cycles  en=off  latency=1  msb_inp=100  msb=100  lsb=-100  use_behavioral_HDL=on  implementation=Fabric  dbl_ovrd=off  block_type=accum
      settings: xl_area=[0, 0, 0, 0, 0, 0, 0]  block_version=10.1.3
  Accumulator1 : xbsIndex_r4/Accumulator  operation=Add  n_bits=32  overflow=Wrap  scale=1  rst=on  hasbypass=on  infoeditControl=reset for floating point data type must be asserted for a minimum of 2 cycles  en=off  latency=1  msb_inp=100  msb=100  lsb=-100  use_behavioral_HDL=on  implementation=Fabric  dbl_ovrd=off  block_type=accum
      settings: xl_area=[0, 0, 0, 0, 0, 0, 0]  block_version=10.1.3
  Accumulator2 : xbsIndex_r4/Accumulator  operation=Add  n_bits=32  overflow=Wrap  scale=1  rst=on  hasbypass=on  infoeditControl=reset for floating point data type must be asserted for a minimum of 2 cycles  en=off  latency=1  msb_inp=100  msb=100  lsb=-100  use_behavioral_HDL=on  implementation=Fabric  dbl_ovrd=off  block_type=accum
      settings: xl_area=[0, 0, 0, 0, 0, 0, 0]  block_version=10.1.3
  BitBasher : xbsIndex_r4/BitBasher  bitexpr=sss={clip, s, ss}  display_expr=off  sr_1=sss  arith_type1="Signed  (2's comp)"  bin_pt1=0  sr_2=2  arith_type2=Unsigned  bin_pt2=0  sr_3=3  arith_type3=Unsigned  bin_pt3=0  sr_4=4  arith_type4=Unsigned  bin_pt4=0  dbl_ovrd=off  block_type=bitbasher
      settings: block_version=10.1.3
  Constant : xbsIndex_r4/Constant  const=127^2  gui_display_data_type=Fixed-point  arith_type=Unsigned  n_bits=15  bin_pt=0  preci_type=Single  exp_width=8  frac_width=24  explicit_period=on  period=1  equ=P=C  opselect=C  inp2=PCIN>>17  opr=+  inp1=P  carry=CIN  dbl_ovrd=off  block_type=constant
  Delay : xbsIndex_r4/Delay  rst=off  infoeditControl=Selection of Reset will increase slice count due to use of real FFs and instead of SRLs  en=off  latency=2  reg_retiming=off  dbl_ovrd=off  block_type=delay
  Delay1 : xbsIndex_r4/Delay  rst=off  infoeditControl=Selection of Reset will increase slice count due to use of real FFs and instead of SRLs  en=off  latency=1  reg_retiming=off  dbl_ovrd=off  block_type=delay
  Delay2 : xbsIndex_r4/Delay  rst=off  infoeditControl=Selection of Reset will increase slice count due to use of real FFs and instead of SRLs  en=off  latency=1  reg_retiming=off  dbl_ovrd=off  block_type=delay
      settings: infoedit=Hardware notes: A delay line is a chain, each link of which is an SRL16 or SRL32 followed by a flip-flop.
  Mult : xbsIndex_r4/Mult  precision=User Defined  arith_type=Unsigned  n_bits=15  bin_pt=0  quantization=Truncate  overflow=Wrap  en=off  latency=2  use_behavioral_HDL=on  opt=Speed  use_embedded=on  optimum_pipeline=on  pipeline=on  dbl_ovrd=off  use_rpm=on  placement_style=Rectangular shape  block_type=mult
      settings: xl_area=[0, 0, 0, 0, 0, 0, 0]  block_version=10.1.3
  Register : xbsIndex_r4/Register  init=0  rst=off  en=on  dbl_ovrd=off  block_type=register
      settings: xl_area=[0, 0, 0, 0, 0, 0, 0]
  Register1 : xbsIndex_r4/Register  init=0  rst=off  en=on  dbl_ovrd=off  block_type=register
      settings: xl_area=[0, 0, 0, 0, 0, 0, 0]
  Register2 : xbsIndex_r4/Register  init=0  rst=off  en=on  dbl_ovrd=off  block_type=register
      settings: xl_area=[0, 0, 0, 0, 0, 0, 0]
  Reinterpret : xbsIndex_r4/Reinterpret  force_arith_type=off  arith_type=Unsigned  force_bin_pt=on  bin_pt=0  block_type=reinterpret
  Relational : xbsIndex_r4/Relational  mode=a>=b  op_type=Ufix  en=off  latency=0  dbl_ovrd=off  block_type=relational
  sum_sumsq : Outport
  wires:
  Register2/1 -> BitBasher/1
  Register/1 -> BitBasher/3
  Register1/1 -> BitBasher/2
  Accumulator2/1 -> Register2/1
  Delay2/1 -> Register/2, Register1/2, Register2/2, Accumulator/2, Accumulator1/2, Accumulator2/2
  Relational/1 -> Accumulator2/1
  Constant/1 -> Relational/2
  Reinterpret/1 -> Delay1/1
  Delay1/1 -> Delay/1, Mult/1, Mult/2
  BitBasher/1 -> sum_sumsq/1
  Delay/1 -> Accumulator1/1
  Accumulator1/1 -> Register1/1
  Mult/1 -> Relational/1, Accumulator/1
  Accumulator/1 -> Register/1
  [adc_rms_rst] -> Delay2/1
  in/1 -> Reinterpret/1

== system snap_sys_clk_feng/stats/calc_adc_sum_sq5 ==
  note: 127^2 == 16129
  in : Inport
  Accumulator : xbsIndex_r4/Accumulator  operation=Add  n_bits=32  overflow=Wrap  scale=1  rst=on  hasbypass=on  infoeditControl=reset for floating point data type must be asserted for a minimum of 2 cycles  en=off  latency=1  msb_inp=100  msb=100  lsb=-100  use_behavioral_HDL=on  implementation=Fabric  dbl_ovrd=off  block_type=accum
      settings: xl_area=[0, 0, 0, 0, 0, 0, 0]  block_version=10.1.3
  Accumulator1 : xbsIndex_r4/Accumulator  operation=Add  n_bits=32  overflow=Wrap  scale=1  rst=on  hasbypass=on  infoeditControl=reset for floating point data type must be asserted for a minimum of 2 cycles  en=off  latency=1  msb_inp=100  msb=100  lsb=-100  use_behavioral_HDL=on  implementation=Fabric  dbl_ovrd=off  block_type=accum
      settings: xl_area=[0, 0, 0, 0, 0, 0, 0]  block_version=10.1.3
  Accumulator2 : xbsIndex_r4/Accumulator  operation=Add  n_bits=32  overflow=Wrap  scale=1  rst=on  hasbypass=on  infoeditControl=reset for floating point data type must be asserted for a minimum of 2 cycles  en=off  latency=1  msb_inp=100  msb=100  lsb=-100  use_behavioral_HDL=on  implementation=Fabric  dbl_ovrd=off  block_type=accum
      settings: xl_area=[0, 0, 0, 0, 0, 0, 0]  block_version=10.1.3
  BitBasher : xbsIndex_r4/BitBasher  bitexpr=sss={clip, s, ss}  display_expr=off  sr_1=sss  arith_type1="Signed  (2's comp)"  bin_pt1=0  sr_2=2  arith_type2=Unsigned  bin_pt2=0  sr_3=3  arith_type3=Unsigned  bin_pt3=0  sr_4=4  arith_type4=Unsigned  bin_pt4=0  dbl_ovrd=off  block_type=bitbasher
      settings: block_version=10.1.3
  Constant : xbsIndex_r4/Constant  const=127^2  gui_display_data_type=Fixed-point  arith_type=Unsigned  n_bits=15  bin_pt=0  preci_type=Single  exp_width=8  frac_width=24  explicit_period=on  period=1  equ=P=C  opselect=C  inp2=PCIN>>17  opr=+  inp1=P  carry=CIN  dbl_ovrd=off  block_type=constant
  Delay : xbsIndex_r4/Delay  rst=off  infoeditControl=Selection of Reset will increase slice count due to use of real FFs and instead of SRLs  en=off  latency=2  reg_retiming=off  dbl_ovrd=off  block_type=delay
  Delay1 : xbsIndex_r4/Delay  rst=off  infoeditControl=Selection of Reset will increase slice count due to use of real FFs and instead of SRLs  en=off  latency=1  reg_retiming=off  dbl_ovrd=off  block_type=delay
  Delay2 : xbsIndex_r4/Delay  rst=off  infoeditControl=Selection of Reset will increase slice count due to use of real FFs and instead of SRLs  en=off  latency=1  reg_retiming=off  dbl_ovrd=off  block_type=delay
      settings: infoedit=Hardware notes: A delay line is a chain, each link of which is an SRL16 or SRL32 followed by a flip-flop.
  Mult : xbsIndex_r4/Mult  precision=User Defined  arith_type=Unsigned  n_bits=15  bin_pt=0  quantization=Truncate  overflow=Wrap  en=off  latency=2  use_behavioral_HDL=on  opt=Speed  use_embedded=on  optimum_pipeline=on  pipeline=on  dbl_ovrd=off  use_rpm=on  placement_style=Rectangular shape  block_type=mult
      settings: xl_area=[0, 0, 0, 0, 0, 0, 0]  block_version=10.1.3
  Register : xbsIndex_r4/Register  init=0  rst=off  en=on  dbl_ovrd=off  block_type=register
      settings: xl_area=[0, 0, 0, 0, 0, 0, 0]
  Register1 : xbsIndex_r4/Register  init=0  rst=off  en=on  dbl_ovrd=off  block_type=register
      settings: xl_area=[0, 0, 0, 0, 0, 0, 0]
  Register2 : xbsIndex_r4/Register  init=0  rst=off  en=on  dbl_ovrd=off  block_type=register
      settings: xl_area=[0, 0, 0, 0, 0, 0, 0]
  Reinterpret : xbsIndex_r4/Reinterpret  force_arith_type=off  arith_type=Unsigned  force_bin_pt=on  bin_pt=0  block_type=reinterpret
  Relational : xbsIndex_r4/Relational  mode=a>=b  op_type=Ufix  en=off  latency=0  dbl_ovrd=off  block_type=relational
  sum_sumsq : Outport
  wires:
  in/1 -> Reinterpret/1
  [adc_rms_rst] -> Delay2/1
  Accumulator/1 -> Register/1
  Mult/1 -> Accumulator/1, Relational/1
  Accumulator1/1 -> Register1/1
  Delay/1 -> Accumulator1/1
  BitBasher/1 -> sum_sumsq/1
  Delay1/1 -> Mult/2, Mult/1, Delay/1
  Reinterpret/1 -> Delay1/1
  Constant/1 -> Relational/2
  Relational/1 -> Accumulator2/1
  Delay2/1 -> Accumulator2/2, Accumulator1/2, Accumulator/2, Register2/2, Register1/2, Register/2
  Accumulator2/1 -> Register2/1
  Register1/1 -> BitBasher/2
  Register/1 -> BitBasher/3
  Register2/1 -> BitBasher/1

== system snap_sys_clk_feng/stats/calc_adc_sum_sq6 ==
  note: 127^2 == 16129
  in : Inport
  Accumulator : xbsIndex_r4/Accumulator  operation=Add  n_bits=32  overflow=Wrap  scale=1  rst=on  hasbypass=on  infoeditControl=reset for floating point data type must be asserted for a minimum of 2 cycles  en=off  latency=1  msb_inp=100  msb=100  lsb=-100  use_behavioral_HDL=on  implementation=Fabric  dbl_ovrd=off  block_type=accum
      settings: xl_area=[0, 0, 0, 0, 0, 0, 0]  block_version=10.1.3
  Accumulator1 : xbsIndex_r4/Accumulator  operation=Add  n_bits=32  overflow=Wrap  scale=1  rst=on  hasbypass=on  infoeditControl=reset for floating point data type must be asserted for a minimum of 2 cycles  en=off  latency=1  msb_inp=100  msb=100  lsb=-100  use_behavioral_HDL=on  implementation=Fabric  dbl_ovrd=off  block_type=accum
      settings: xl_area=[0, 0, 0, 0, 0, 0, 0]  block_version=10.1.3
  Accumulator2 : xbsIndex_r4/Accumulator  operation=Add  n_bits=32  overflow=Wrap  scale=1  rst=on  hasbypass=on  infoeditControl=reset for floating point data type must be asserted for a minimum of 2 cycles  en=off  latency=1  msb_inp=100  msb=100  lsb=-100  use_behavioral_HDL=on  implementation=Fabric  dbl_ovrd=off  block_type=accum
      settings: xl_area=[0, 0, 0, 0, 0, 0, 0]  block_version=10.1.3
  BitBasher : xbsIndex_r4/BitBasher  bitexpr=sss={clip, s, ss}  display_expr=off  sr_1=sss  arith_type1="Signed  (2's comp)"  bin_pt1=0  sr_2=2  arith_type2=Unsigned  bin_pt2=0  sr_3=3  arith_type3=Unsigned  bin_pt3=0  sr_4=4  arith_type4=Unsigned  bin_pt4=0  dbl_ovrd=off  block_type=bitbasher
      settings: block_version=10.1.3
  Constant : xbsIndex_r4/Constant  const=127^2  gui_display_data_type=Fixed-point  arith_type=Unsigned  n_bits=15  bin_pt=0  preci_type=Single  exp_width=8  frac_width=24  explicit_period=on  period=1  equ=P=C  opselect=C  inp2=PCIN>>17  opr=+  inp1=P  carry=CIN  dbl_ovrd=off  block_type=constant
  Delay : xbsIndex_r4/Delay  rst=off  infoeditControl=Selection of Reset will increase slice count due to use of real FFs and instead of SRLs  en=off  latency=2  reg_retiming=off  dbl_ovrd=off  block_type=delay
  Delay1 : xbsIndex_r4/Delay  rst=off  infoeditControl=Selection of Reset will increase slice count due to use of real FFs and instead of SRLs  en=off  latency=1  reg_retiming=off  dbl_ovrd=off  block_type=delay
  Delay2 : xbsIndex_r4/Delay  rst=off  infoeditControl=Selection of Reset will increase slice count due to use of real FFs and instead of SRLs  en=off  latency=1  reg_retiming=off  dbl_ovrd=off  block_type=delay
      settings: infoedit=Hardware notes: A delay line is a chain, each link of which is an SRL16 or SRL32 followed by a flip-flop.
  Mult : xbsIndex_r4/Mult  precision=User Defined  arith_type=Unsigned  n_bits=15  bin_pt=0  quantization=Truncate  overflow=Wrap  en=off  latency=2  use_behavioral_HDL=on  opt=Speed  use_embedded=on  optimum_pipeline=on  pipeline=on  dbl_ovrd=off  use_rpm=on  placement_style=Rectangular shape  block_type=mult
      settings: xl_area=[0, 0, 0, 0, 0, 0, 0]  block_version=10.1.3
  Register : xbsIndex_r4/Register  init=0  rst=off  en=on  dbl_ovrd=off  block_type=register
      settings: xl_area=[0, 0, 0, 0, 0, 0, 0]
  Register1 : xbsIndex_r4/Register  init=0  rst=off  en=on  dbl_ovrd=off  block_type=register
      settings: xl_area=[0, 0, 0, 0, 0, 0, 0]
  Register2 : xbsIndex_r4/Register  init=0  rst=off  en=on  dbl_ovrd=off  block_type=register
      settings: xl_area=[0, 0, 0, 0, 0, 0, 0]
  Reinterpret : xbsIndex_r4/Reinterpret  force_arith_type=off  arith_type=Unsigned  force_bin_pt=on  bin_pt=0  block_type=reinterpret
  Relational : xbsIndex_r4/Relational  mode=a>=b  op_type=Ufix  en=off  latency=0  dbl_ovrd=off  block_type=relational
  sum_sumsq : Outport
  wires:
  in/1 -> Reinterpret/1
  [adc_rms_rst] -> Delay2/1
  Accumulator/1 -> Register/1
  Mult/1 -> Accumulator/1, Relational/1
  Accumulator1/1 -> Register1/1
  Delay/1 -> Accumulator1/1
  BitBasher/1 -> sum_sumsq/1
  Delay1/1 -> Mult/2, Mult/1, Delay/1
  Reinterpret/1 -> Delay1/1
  Constant/1 -> Relational/2
  Relational/1 -> Accumulator2/1
  Delay2/1 -> Accumulator2/2, Accumulator1/2, Accumulator/2, Register2/2, Register1/2, Register/2
  Accumulator2/1 -> Register2/1
  Register1/1 -> BitBasher/2
  Register/1 -> BitBasher/3
  Register2/1 -> BitBasher/1
